simulink model "invertor_basic_model1"  (R2025a)
settings: Solver=ode45  StartTime=0.0  StopTime=0.1  MaxStep=1e-7  MinStep=1e-8  RelTol=1e-3
libraries: spsMosfetLib x4, spsSeriesRLCBranchLib x3, spsCurrentMeasurementLib x1, spsDCVoltageSourceLib x1, simulink x1, spsVoltageMeasurementLib x1, sps_lib x1
settings Model: Creator=Kamal Dhali  LastModifiedBy=Kamal Dhali

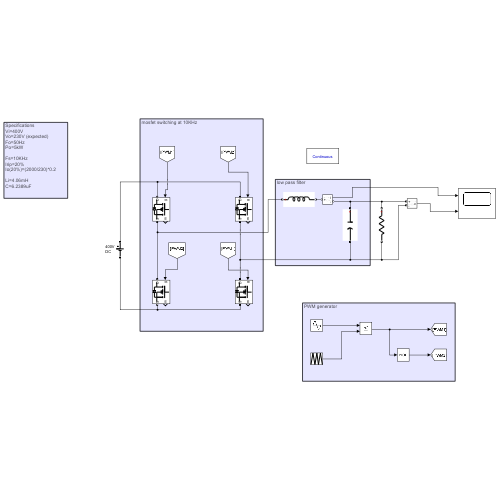
[thumbnail: Simulink's stored preview of the top-level diagram]
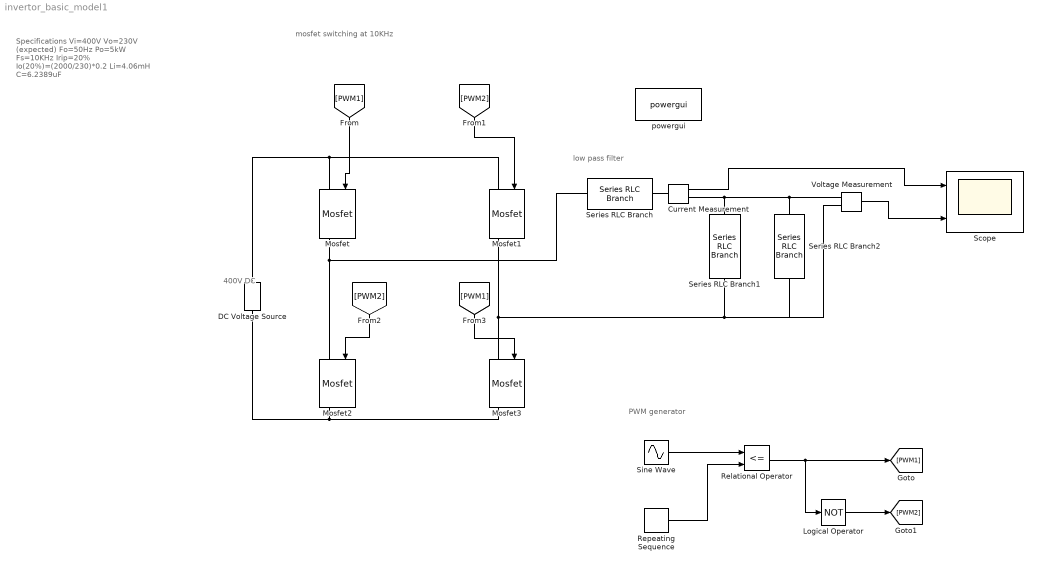
== system invertor_basic_model1 ==
  note: 400V
      | DC
  note: Specifications
      | Vi=400V
      | Vo=230V (expected)
      | Fo=50Hz
      | Po=5kW
      |
      | Fs=10KHz
      | Irip=20%
      | Io(20%)=(2000/230)*0.2
      |
      | Li=4.06mH
      | C=6.2389uF
  note: low pass filter
  note: mosfet switching at 10KHz
  note: PWM generator
  Current Measurement : spsCurrentMeasurementLib/Current Measurement  PhasorSimulation=off  OutputType=Complex  PSBequivalent=0
  DC Voltage Source : spsDCVoltageSourceLib/DC Voltage Source  Amplitude=400  Measurements=None
  Logical Operator : Logic  Operator=NOT  AllPortsSameDT=off  OutDataTypeStr=boolean
  Mosfet{,1..3} (4 alike) : spsMosfetLib/Mosfet  Ron=0.1  Lon=0  Rd=0.01  Vfd=0  IC=0  Rs=1e5  Cs=inf  Measurements=on
  Relational Operator : RelationalOperator  Operator=<=  OutDataTypeStr=boolean  RndMeth=Simplest  InputSameDT=off
  Repeating Sequence : simulink/Sources/Repeating Sequence  rep_seq_t=[0 0.00005 0.0001]  rep_seq_y=[-1 1 -1]
  Scope : Scope  NumInputPorts=2
      settings: ActiveDisplayYMinimum=-865.81395003345835  ActiveDisplayYMaximum=1154.6502993590882
  Series RLC Branch : spsSeriesRLCBranchLib/Series RLC Branch  LConnTagsString=__new0  RConnTagsString=__new0  BranchType=L  Resistance=1  Inductance=4.06e-3  SetiL0=off  InitialCurrent=0  Capacitance=1e-6  Setx0=off  InitialVoltage=0  Measurements=None
  Series RLC Branch1 : spsSeriesRLCBranchLib/Series RLC Branch  LConnTagsString=__new0  RConnTagsString=__new0  BranchType=C  Resistance=1  Inductance=1e-3  SetiL0=off  InitialCurrent=0  Capacitance=6.2389e-6  Setx0=off  InitialVoltage=0  Measurements=None
  Series RLC Branch2 : spsSeriesRLCBranchLib/Series RLC Branch  LConnTagsString=__new0  RConnTagsString=__new0  BranchType=R  Resistance=100  Inductance=1e-3  SetiL0=off  InitialCurrent=0  Capacitance=1e-6  Setx0=off  InitialVoltage=0  Measurements=None
  Sine Wave : Sin  Amplitude=0.45  Frequency=2*pi*50  SampleTime=0
  Voltage Measurement : spsVoltageMeasurementLib/Voltage Measurement  PhasorSimulation=off  OutputType=Complex  PSBequivalent=0
  powergui : sps_lib/powergui  Priority=1  SimulationMode=Continuous  SampleTime=50e-6  frequency=60  Iterations=50  frequencyindice=0  Pbase=100e6  ErrMax=1e-4  UnitsV=kV  UnitsW=MW  buscounter=0  FunctionMessages=off  echomessages=off  EnableUseOfTLC=off  CurrentSourceSwitches=off  DisableSnubberDevices=off  DisableRonSwitches=off  DisableVfSwitches=off  DisplayEquations=off  AutomaticDiscreteSolvers=off  SolverType=Tustin/Backward Euler (TBE)  Interpol=off  ExternalGateDelay=off  methode=off  Ts=100  x0status=blocks  SPID=on  SwTol=0  HookPort=off  NonlinearTolerance=1e-4  nMaxIteration=100  ContinueOnMaxIteration=off  RestoreLinks=warning  ResistiveCurrentMeasurement=off  Frange=[0:2:500]  Ylog=off  Xlog=on  ShowGrid=off  save=off  variable=ZData  structure=0  ZoomFFT=off  StartTime=0.0  cycles=1  DisplayStyle=1  fundamental=60  FreqAxis=off  MaxFrequency=1000  frequencyindicesteady=1  RmsSteady=1  display=off
  wires:
  Voltage Measurement/1 -> Scope/2
  Repeating Sequence/1 -> Relational Operator/2
  Sine Wave/1 -> Relational Operator/1
  Relational Operator/1 -> [PWM1], Logical Operator/1
  Logical Operator/1 -> [PWM2]
  Current Measurement/1 -> Scope/1
  [PWM1] -> Mosfet/1
  [PWM2] -> Mosfet2/1
  [PWM2] -> Mosfet1/1
  [PWM1] -> Mosfet3/1
  connections:
  Mosfet/RConn1 -- Mosfet2/LConn1 -- Series RLC Branch/LConn1
  Mosfet3/LConn1 -- Voltage Measurement/LConn2 -- Series RLC Branch2/RConn1 -- Series RLC Branch1/RConn1 -- Mosfet1/RConn1
  Mosfet/LConn1 -- DC Voltage Source/RConn1 -- Mosfet1/LConn1
  Mosfet2/RConn1 -- Mosfet3/RConn1 -- DC Voltage Source/LConn1
  Current Measurement/LConn1 -- Series RLC Branch/RConn1
  Current Measurement/RConn1 -- Voltage Measurement/LConn1 -- Series RLC Branch2/LConn1 -- Series RLC Branch1/LConn1
